simulink library "Lib_Piccolo"  (R2018b)
settings: Solver=VariableStepAuto  StartTime=0.0  StopTime=10.0  RelTol=1e-3
values from neighbouring files (symbols this model uses):
  AccelErrInt2Brakes = 0.15    [SimulationControlConfig16P.m]    (also in SimulationControlConfig16P_LEGACY.m; SimulationControlConfigTAILLESS.m = 0.2; SimulationControlConfigUTAIL.m = 0.2)
  AileronMax = 25    [SimulationControlConfig16P.m]    (also in SimulationControlConfig16P_LEGACY.m; SimulationControlConfigTAILLESS.m; SimulationControlConfigUTAIL.m)
  AileronPower = 0.00268    [SimulationControlConfig16P.m]    (also in SimulationControlConfig16P_LEGACY.m; SimulationControlConfigTAILLESS.m; SimulationControlConfigUTAIL.m)
  AileronSurfaceMax = 45    [SimulationControlConfig16P.m]    (also in SimulationControlConfig16P_LEGACY.m)
  AileronTrim = 0    [SimulationControlConfig16P.m]    (also in SimulationControlConfig16P_LEGACY.m; SimulationControlConfigTAILLESS.m; SimulationControlConfigUTAIL.m)
  Alt = 1000 + TerrainHeight    [SimulationStateConfig.m]
  AltCruise_m = testPlans(testIndx).terrainElevation * 0.3048 + 200    [SimulationControlConfig16P.m]    (also in SimulationControlConfigTAILLESS.m = 1083; SimulationControlConfigUTAIL.m = testPlans(testIndx).terrainElevation * 0.3048 + 152)
  AltitudeRate2PitchCmdIntegratorInit = 0.1    [SimulationControlPre.m]
  AltMax = 10000    [SimulationControlConfig16P.m]    (also in SimulationControlConfig16P_LEGACY.m; SimulationControlConfigTAILLESS.m; SimulationControlConfigUTAIL.m)
  AltMaxAccel = 1.25    [SimulationControlConfig16P.m]    (also in SimulationControlConfig16P_LEGACY.m = 0.9; SimulationControlConfigTAILLESS.m = 1.7; SimulationControlConfigUTAIL.m = 2)
  AltMin = 0    [SimulationControlConfig16P.m]    (also in SimulationControlConfig16P_LEGACY.m; SimulationControlConfigTAILLESS.m; SimulationControlConfigUTAIL.m)
  AltRateCmd2Pitch = 0.50    (= 0.5)    [SimulationControlConfig16P.m]    (also in SimulationControlConfig16P_LEGACY.m = 0.6; SimulationControlConfigTAILLESS.m = 0.2; SimulationControlConfigUTAIL.m = 0.3)
  AltRateError2Pitch = 0.40    (= 0.4)    [SimulationControlConfig16P.m]    (also in SimulationControlConfig16P_LEGACY.m; SimulationControlConfigTAILLESS.m = 0.55; SimulationControlConfigUTAIL.m = 0.55)
  AltRateErrorInt2Pitch = 0.50    (= 0.5)    [SimulationControlConfig16P.m]    (also in SimulationControlConfig16P_LEGACY.m = 0.45; SimulationControlConfigTAILLESS.m; SimulationControlConfigUTAIL.m = 0.75)
  AltRateLpfCutOff = 3    [SimulationControlConfig16P.m]    (also in SimulationControlConfig16P_LEGACY.m; SimulationControlConfigTAILLESS.m = 2; SimulationControlConfigUTAIL.m = 2)
  AutoNosegear2Rudder = 26    [SimulationControlConfig16P.m]    (also in SimulationControlConfig16P_LEGACY.m; SimulationControlConfigTAILLESS.m = 25.2; SimulationControlConfigUTAIL.m = 14)
  b = 5.54    [SimulationControlConfig16P.m]    (also in SimulationControlConfig16P_LEGACY.m; SimulationControlConfigTAILLESS.m = 2.37; SimulationControlConfigUTAIL.m = 2.37)
  Bank2AileronIntegratorInit = 0    [SimulationControlPre.m]
  BankMax_User = BankMax_User/180*pi    (= 0.523598775598)    [SimulationControlConfig16P.m]    (also in SimulationControlConfig16P_LEGACY.m; SimulationControlConfigTAILLESS.m = 0.610865238198; SimulationControlConfigUTAIL.m = 0.628318530718)
  baseLegFlaps = 20    [SimulationControlConfig16P.m]    (also in SimulationControlConfig16P_LEGACY.m = 0; SimulationControlConfigTAILLESS.m = 15; SimulationControlConfigUTAIL.m = 10)
  C = GeneticOpt.C    [SimulationCostFunction.m]
  c = Sw/b    (= 0.841696750903)    [SimulationControlConfig16P.m]    (also in SimulationControlConfig16P_LEGACY.m; SimulationControlConfigTAILLESS.m = 0.354008438819; SimulationControlConfigUTAIL.m = 0.354008438819)
  cell2WheelFactorMG = 5.98    [SimulationSensorConfig16P_LEGACY.m]
  cell2WheelFactorNG = 1    [SimulationSensorConfig16P_LEGACY.m]
  cellSatMaxMG = 15000    [SimulationSensorConfig16P.m]    (also in SimulationSensorConfig16P_LEGACY.m; SimulationSensorConfigTAILLESS7P.m; SimulationSensorConfigUTAIL7P.m)
  cellSatMaxNG = 1000    [SimulationSensorConfig16P.m]    (also in SimulationSensorConfig16P_LEGACY.m; SimulationSensorConfigTAILLESS7P.m; SimulationSensorConfigUTAIL7P.m)
  cellSatMinMG = -15000    [SimulationSensorConfig16P.m]    (also in SimulationSensorConfig16P_LEGACY.m; SimulationSensorConfigTAILLESS7P.m; SimulationSensorConfigUTAIL7P.m)
  cellSatMinNG = -1000    [SimulationSensorConfig16P.m]    (also in SimulationSensorConfig16P_LEGACY.m; SimulationSensorConfigTAILLESS7P.m; SimulationSensorConfigUTAIL7P.m)
  CL_Limit = CL_Max    (= 0.54)    [SimulationControlConfig16P.m]    (also in SimulationControlConfig16P_LEGACY.m; SimulationControlConfigTAILLESS.m; SimulationControlConfigUTAIL.m = 0.53)
  CL_Max = 0.54    [SimulationControlConfig16P.m]    (also in SimulationControlConfig16P_LEGACY.m; SimulationControlConfigTAILLESS.m; SimulationControlConfigUTAIL.m = 0.53)
  CL_Max_Nom = 0.465    [SimulationControlConfig16P.m]    (also in SimulationControlConfig16P_LEGACY.m; SimulationControlConfigTAILLESS.m = 0.39; SimulationControlConfigUTAIL.m)
  CL_Min = 0    [SimulationControlConfig16P.m]    (also in SimulationControlConfig16P_LEGACY.m; SimulationControlConfigTAILLESS.m; SimulationControlConfigUTAIL.m)
  ClimbMaxFraction = 0.35    [SimulationControlConfig16P.m]    (also in SimulationControlConfig16P_LEGACY.m = 0.24; SimulationControlConfigTAILLESS.m = 0.19; SimulationControlConfigUTAIL.m = 0.21)
  ClimboutMaxBank = 7.0    (= 7)    [SimulationControlConfig16P.m]    (also in SimulationControlConfig16P_LEGACY.m; SimulationControlConfigTAILLESS.m = 5; SimulationControlConfigUTAIL.m)
  ClimboutTimer = 7.0    (= 7)    [SimulationControlConfig16P.m]    (also in SimulationControlConfig16P_LEGACY.m; SimulationControlConfigTAILLESS.m; SimulationControlConfigUTAIL.m)
  dCl_per_dFlap = 0.005581818    [SimulationControlConfig16P.m]    (also in SimulationControlConfig16P_LEGACY.m = 0; SimulationControlConfigTAILLESS.m = 0; SimulationControlConfigUTAIL.m = 0)
  DecelerationCmd = 3.1    [SimulationControlConfig16P.m]    (also in SimulationControlConfig16P_LEGACY.m; SimulationControlConfigTAILLESS.m = 0.1; SimulationControlConfigUTAIL.m = 0.1)
  DeRotateLogicEndTimer = abs((NoseDownLimit_Deg-1)/DeRotateRamp_Dps)    [SimulationControlConfig16P.m]    (also in SimulationControlConfig16P_LEGACY.m; SimulationControlConfigTAILLESS.m; SimulationControlConfigUTAIL.m)
  DeRotateLogicHoldNoseUpTimer = 0.1    [SimulationControlConfig16P.m]    (also in SimulationControlConfig16P_LEGACY.m; SimulationControlConfigTAILLESS.m; SimulationControlConfigUTAIL.m)
  DeRotateLogicTimerTimeout = 2    [SimulationControlConfig16P.m]    (also in SimulationControlConfig16P_LEGACY.m; SimulationControlConfigTAILLESS.m; SimulationControlConfigUTAIL.m)
  DeRotateLowerCmdSaturation = 0    [SimulationControlConfig16P.m]    (also in SimulationControlConfig16P_LEGACY.m; SimulationControlConfigTAILLESS.m; SimulationControlConfigUTAIL.m)
  DeRotateRamp_Dps = 3    [SimulationControlConfig16P.m]    (also in SimulationControlConfig16P_LEGACY.m; SimulationControlConfigTAILLESS.m = 8; SimulationControlConfigUTAIL.m = 8)
  DeRotateUpperCmdSaturation = 7    [SimulationControlConfig16P.m]    (also in SimulationControlConfig16P_LEGACY.m; SimulationControlConfigTAILLESS.m; SimulationControlConfigUTAIL.m)
  DescentMaxFraction = 0.22    [SimulationControlConfig16P.m]    (also in SimulationControlConfig16P_LEGACY.m = 0.2; SimulationControlConfigTAILLESS.m = 0.17; SimulationControlConfigUTAIL.m = 0.17)
  DesktopSimTerrainOffset_m = 0.406    [SimulationAircraftConfig.m]
  downwindFlaps = 0    [SimulationControlConfig16P.m]    (also in SimulationControlConfig16P_LEGACY.m; SimulationControlConfigTAILLESS.m; SimulationControlConfigUTAIL.m)
  DP_init = 0.5*1.225*V_init^2    [SimulationControlConfig16P.m]    (also in SimulationControlConfig16P_LEGACY.m; SimulationControlConfigTAILLESS.m; SimulationControlConfigUTAIL.m)
  dscNoiseMG = 1    [SimulationSensorConfig16P_LEGACY.m]
  dscNoiseNG = 0.25    [SimulationSensorConfig16P_LEGACY.m]
  DSCnumBits = 24    [SimulationSensorConfig16P.m]    (also in SimulationSensorConfig16P_LEGACY.m; SimulationSensorConfigTAILLESS7P.m; SimulationSensorConfigUTAIL7P.m)
  DSCRangeMaxMG = 15000    [SimulationSensorConfig16P.m]    (also in SimulationSensorConfig16P_LEGACY.m; SimulationSensorConfigTAILLESS7P.m; SimulationSensorConfigUTAIL7P.m)
  DSCRangeMaxNG = 1000    [SimulationSensorConfig16P.m]    (also in SimulationSensorConfig16P_LEGACY.m; SimulationSensorConfigTAILLESS7P.m; SimulationSensorConfigUTAIL7P.m)
  DSCRangeMinMG = -15000    [SimulationSensorConfig16P.m]    (also in SimulationSensorConfig16P_LEGACY.m; SimulationSensorConfigTAILLESS7P.m; SimulationSensorConfigUTAIL7P.m)
  DSCRangeMinNG = -1000    [SimulationSensorConfig16P.m]    (also in SimulationSensorConfig16P_LEGACY.m; SimulationSensorConfigTAILLESS7P.m; SimulationSensorConfigUTAIL7P.m)
  dt = DLLSim.dt    [SimulationTimeStep.m]    (also in SimulationTrim.m = 0.02)
  EarlyTouchdownThreshold = 3.0    (= 3)    [SimulationControlConfig16P.m]    (also in SimulationControlConfig16P_LEGACY.m; SimulationControlConfigTAILLESS.m = 2.2; SimulationControlConfigUTAIL.m = 2.5)
  ElevatorDeflectionRate = 15    [SimulationControlConfig16P.m]    (also in SimulationControlConfig16P_LEGACY.m = 12; SimulationControlConfigTAILLESS.m = 10; SimulationControlConfigUTAIL.m = 12)
  ElevatorMax = 25    [SimulationControlConfig16P.m]    (also in SimulationControlConfig16P_LEGACY.m; SimulationControlConfigTAILLESS.m; SimulationControlConfigUTAIL.m)
  ElevatorPower = -0.002209    [SimulationControlConfig16P.m]    (also in SimulationControlConfig16P_LEGACY.m; SimulationControlConfigTAILLESS.m = -0.002956; SimulationControlConfigUTAIL.m = -0.00205983)
  ElevatorTrim = -3.5    [SimulationControlConfig16P.m]    (also in SimulationControlConfig16P_LEGACY.m; SimulationControlConfigTAILLESS.m = -6; SimulationControlConfigUTAIL.m = -8)
  elevonBias = 0    [SimulationControlConfig16P.m]    (also in SimulationControlConfig16P_LEGACY.m; SimulationControlConfigTAILLESS.m; SimulationControlConfigUTAIL.m)
  Enable_TAS_Protection = 0    [SimulationControlConfig16P.m]    (also in SimulationControlConfig16P_LEGACY.m; SimulationControlConfigTAILLESS.m; SimulationControlConfigUTAIL.m)
  EnableCrossTrackAbort = 1    [SimulationControlConfig16P.m]    (also in SimulationControlConfigTAILLESS.m; SimulationControlConfigUTAIL.m)
  EnergyBandwidth = 0.02    [SimulationControlConfig16P.m]    (also in SimulationControlConfig16P_LEGACY.m; SimulationControlConfigTAILLESS.m = 0.06; SimulationControlConfigUTAIL.m = 0.06)
  EngineLhFuelCut = 0    [SimulationAircraftConfig.m]
  EngineRhFuelCut = 0    [SimulationAircraftConfig.m]
  FastThrottleRate = 0.075    [SimulationControlConfig16P.m]    (also in SimulationControlConfig16P_LEGACY.m = 0.05; SimulationControlConfigTAILLESS.m = 0.1; SimulationControlConfigUTAIL.m = 0.1)
  FilterWarmUpTime = 2    [SimulationSensorConfig16P.m]    (also in SimulationSensorConfig16P_LEGACY.m; SimulationSensorConfigTAILLESS7P.m; SimulationSensorConfigUTAIL7P.m)
  finalApproachFlaps = 20    [SimulationControlConfig16P.m]    (also in SimulationControlConfig16P_LEGACY.m = 0; SimulationControlConfigTAILLESS.m = 22; SimulationControlConfigUTAIL.m = 10)
  FinalDescentSlope_Deg = testPlans(testIndx).descentSlope    [SimulationControlConfig16P.m]    (also in SimulationControlConfig16P_LEGACY.m; SimulationControlConfigTAILLESS.m; SimulationControlConfigUTAIL.m)
  flapMax = 0    [SimulationControlConfig16P.m]    (also in SimulationControlConfig16P_LEGACY.m; SimulationControlConfigTAILLESS.m; SimulationControlConfigUTAIL.m)
  flapRate = 7.5    [SimulationControlConfig16P.m]    (also in SimulationControlConfig16P_LEGACY.m; SimulationControlConfigTAILLESS.m = 6.6; SimulationControlConfigUTAIL.m)
  FlareHeight = 5    [SimulationControlConfig16P.m]    (also in SimulationControlConfig16P_LEGACY.m = 4.8; SimulationControlConfigTAILLESS.m = 2.5; SimulationControlConfigUTAIL.m = 2)
  FlareVerticalRate_mps = -0.4    [SimulationControlConfig16P.m]    (also in SimulationControlConfig16P_LEGACY.m = -0.5; SimulationControlConfigTAILLESS.m = -0.15; SimulationControlConfigUTAIL.m = -0.15)
  Fp_Aileron = 0.55*2*pi*RollRateLpfCutoff*dt    [SimulationControlConfig16P.m]    (also in SimulationControlConfig16P_LEGACY.m; SimulationControlConfigTAILLESS.m; SimulationControlConfigUTAIL.m)
  Fp_Alt = 0.55*AltBandwidth    (= 0.099)    [SimulationControlConfig16P.m]    (also in SimulationControlConfig16P_LEGACY.m; SimulationControlConfigTAILLESS.m = 0.587477826221; SimulationControlConfigUTAIL.m = 0.69115038379)
  Fp_AltRate = 0.55*2*pi*AltRateLpfCutOff*dt    [SimulationControlConfig16P.m]    (also in SimulationControlConfig16P_LEGACY.m; SimulationControlConfigTAILLESS.m; SimulationControlConfigUTAIL.m)
  Fp_Elevator = 0.55*2*pi*PitchRateLpfCutoff*dt    [SimulationControlConfig16P.m]    (also in SimulationControlConfig16P_LEGACY.m; SimulationControlConfigTAILLESS.m; SimulationControlConfigUTAIL.m)
  Fp_Energy = 0.55*2*pi*EnergyBandwidth    (= 0.069115038379)    [SimulationControlConfig16P.m]    (also in SimulationControlConfig16P_LEGACY.m; SimulationControlConfigTAILLESS.m = 0.207345115137; SimulationControlConfigUTAIL.m = 0.207345115137)
  Fp_Energy2 = 0.55*2*pi*EnergyBandwidth*dt    [SimulationControlConfig16P.m]    (also in SimulationControlConfig16P_LEGACY.m; SimulationControlConfigTAILLESS.m; SimulationControlConfigUTAIL.m)
  Fp_Pitch = 0.55*2*pi*PitchBandwidth    (= 2.76460153516)    [SimulationControlConfig16P.m]    (also in SimulationControlConfig16P_LEGACY.m = 3.11017672705; SimulationControlConfigTAILLESS.m = 3.80132711084; SimulationControlConfigUTAIL.m = 2.41902634326)
  Fp_Pitch_2 = 0.55*2*pi*PitchBandwidth*dt    [SimulationControlConfig16P.m]    (also in SimulationControlConfig16P_LEGACY.m; SimulationControlConfigTAILLESS.m; SimulationControlConfigUTAIL.m)
  Fp_Roll = RollBandwidth^2    (= 1)    [SimulationControlConfig16P.m]    (also in SimulationControlConfig16P_LEGACY.m = 1.44; SimulationControlConfigTAILLESS.m; SimulationControlConfigUTAIL.m)
  Fp_Rudder = 0.55*2*pi*YawRateLpfCutoff*dt    [SimulationControlConfig16P.m]    (also in SimulationControlConfig16P_LEGACY.m; SimulationControlConfigTAILLESS.m; SimulationControlConfigUTAIL.m)
  Fp_TAS = 0.55*2*pi*TASBandwidth    (= 0.103672557568)    [SimulationControlConfig16P.m]    (also in SimulationControlConfig16P_LEGACY.m; SimulationControlConfigTAILLESS.m = 0.172787595947; SimulationControlConfigUTAIL.m = 0.172787595947)
  Fp_TAS_Filter = 2*pi*TasLpfCutoff*dt    [SimulationControlConfig16P.m]    (also in SimulationControlConfig16P_LEGACY.m; SimulationControlConfigTAILLESS.m; SimulationControlConfigUTAIL.m)
  Fp_Turn = 0.55*2*pi*TurnErrLPFcutoff    (= 0.0345575191895)    [SimulationControlConfig16P.m]    (also in SimulationControlConfig16P_LEGACY.m; SimulationControlConfigTAILLESS.m = 0.172787595947; SimulationControlConfigUTAIL.m = 0.172787595947)
  Fp_TurnDerr = 0.55*2*pi*TurnDerivativeLPFcutoff    (= 0.0345575191895)    [SimulationControlConfig16P.m]    (also in SimulationControlConfig16P_LEGACY.m; SimulationControlConfigTAILLESS.m = 0.172787595947; SimulationControlConfigUTAIL.m = 0.172787595947)
  FTV = 3    [SimulationAircraftConfig.m]
  ftvStaticPositionError = 1/1.18    (= 0.847457627119)    [SimulationSensorConfig16P.m]    (also in SimulationSensorConfig16P_LEGACY.m; SimulationSensorConfigTAILLESS7P.m = 1; SimulationSensorConfigUTAIL7P.m = 1)
  g = 9.81    [SimulationStateConfig.m]
  GustSpd_Kts = testPlans(testIndx).gustSpd    [SimulationStateConfig.m]
  GustTriggerVal = testPlans(testIndx).gustTriggerVal    [SimulationStateConfig.m]
  HeadingErr2TurnRate = 0.5    [SimulationControlConfig16P.m]    (also in SimulationControlConfig16P_LEGACY.m; SimulationControlConfigTAILLESS.m; SimulationControlConfigUTAIL.m)
  HeadingErrDer2TurnRate = 0.3    [SimulationControlConfig16P.m]    (also in SimulationControlConfig16P_LEGACY.m; SimulationControlConfigTAILLESS.m; SimulationControlConfigUTAIL.m)
  IASbounce = IASstall*0.8    [SimulationControlPre.m]
  IAScruiseCMD = sqrt(2*m*9.81/(1.225*Sw*CL_cruise))    [SimulationControlConfig16P.m]    (also in SimulationControlConfig16P_LEGACY.m; SimulationControlConfigTAILLESS.m; SimulationControlConfigUTAIL.m)
  IASfinalCMD = 1.12 * IASmin    [SimulationControlConfig16P.m]    (also in SimulationControlConfig16P_LEGACY.m = 1.10 * IASmin; SimulationControlConfigTAILLESS.m = 1.10 * IASmin; SimulationControlConfigUTAIL.m = 1.15 * IASmin)
  IASflareCMD = IASstall    [SimulationControlConfig16P.m]    (also in SimulationControlConfig16P_LEGACY.m; SimulationControlConfigTAILLESS.m; SimulationControlConfigUTAIL.m)
  IASmax = 64    [SimulationControlConfig16P.m]    (also in SimulationControlConfig16P_LEGACY.m = 46; SimulationControlConfigTAILLESS.m = 38.58; SimulationControlConfigUTAIL.m = 35)
  IASmin = sqrt(2*m*9.81/(1.225*Sw*0.9*CL_Max_Nom))    [SimulationControlConfig16P.m]    (also in SimulationControlConfig16P_LEGACY.m; SimulationControlConfigTAILLESS.m; SimulationControlConfigUTAIL.m)
  IASshortCMD = IASstall    [SimulationControlConfig16P.m]    (also in SimulationControlConfig16P_LEGACY.m; SimulationControlConfigTAILLESS.m; SimulationControlConfigUTAIL.m)
  IASstall = sqrt(2*m*9.81/(1.225*Sw*CL_Max))    [SimulationControlConfig16P.m]    (also in SimulationControlConfig16P_LEGACY.m; SimulationControlConfigTAILLESS.m; SimulationControlConfigUTAIL.m)
  inFlight = 1    [SimulationControlConfig16P.m]    (also in SimulationControlConfigTAILLESS.m; SimulationControlConfigUTAIL.m)
  JetCatOffset = 5    [SimulationControlConfig16P.m]    (also in SimulationControlConfig16P_LEGACY.m)
  LaunchRollingElevator = -1.5    [SimulationControlConfig16P.m]    (also in SimulationControlConfig16P_LEGACY.m; SimulationControlConfigTAILLESS.m = 1; SimulationControlConfigUTAIL.m = 1)
  ldg_NosegearMax = 10    [SimulationControlConfig16P.m]    (also in SimulationControlConfig16P_LEGACY.m; SimulationControlConfigTAILLESS.m; SimulationControlConfigUTAIL.m)
  ldg_TrackVyErrInt2Nosegear = 0.1250    (= 0.125)    [SimulationControlConfig16P.m]    (also in SimulationControlConfig16P_LEGACY.m; SimulationControlConfigTAILLESS.m = 0.00714285714286; SimulationControlConfigUTAIL.m = 0.00714285714286)
  ldg_TrackVyErrPro2Nosegear = 0.35    [SimulationControlConfig16P.m]    (also in SimulationControlConfig16P_LEGACY.m; SimulationControlConfigTAILLESS.m = 0.0546666666667; SimulationControlConfigUTAIL.m = 0.0546666666667)
  ldg_TrackY2Vy = 0.07    [SimulationControlConfig16P.m]    (also in SimulationControlConfig16P_LEGACY.m; SimulationControlConfigTAILLESS.m = 0.17; SimulationControlConfigUTAIL.m = 0.17)
  ldg_Vy2NosegearScalingPower = 1.075    [SimulationControlConfig16P.m]    (also in SimulationControlConfig16P_LEGACY.m; SimulationControlConfigTAILLESS.m = 0.6; SimulationControlConfigUTAIL.m = 0.5)
  ldg_Y2VyScalingPower = 0.175    [SimulationControlConfig16P.m]    (also in SimulationControlConfig16P_LEGACY.m; SimulationControlConfigTAILLESS.m = 0; SimulationControlConfigUTAIL.m = 0)
  ldg_YawRate2Nosegear = 0.175    [SimulationControlConfig16P.m]    (also in SimulationControlConfig16P_LEGACY.m; SimulationControlConfigTAILLESS.m = 0.065; SimulationControlConfigUTAIL.m = 0.065)
  LiftSlope = 0.064285    [SimulationControlConfig16P.m]    (also in SimulationControlConfig16P_LEGACY.m; SimulationControlConfigTAILLESS.m = 0.058631; SimulationControlConfigUTAIL.m)
  LPFaileronInit = 0    [SimulationControlPre.m]
  LPFclestInit = 0    [SimulationControlPre.m]
  LPFenergyFFInit = 0    [SimulationControlPre.m]
  LPFtasInit = V_init + 2    [SimulationControlPre.m]
  LPFthrottleInit = ThrottleTrim    [SimulationControlPre.m]
  LPFturnErrInit = 0    [SimulationControlPre.m]
  ... (+115 more)
undefined symbols (not defined in the file or in its folder): abortFlag, alphaHPF, apmDelay, BRWNOUT, CRAWOR, CRAWUR, DiscIntNeverNeededParam, DLLSim, DLLSimStep, ECOMOR, ECOMUR, Fp_Tas, GustTrigger_HeightAgl_m, IPSTAT, LCINTEG, Ldg_Persist_Time, LOWER_FLAGS, MSG_ENABLE, NoiseStd, OLDVAL, OVERRIDE_ENABLE, OVERRIDE_VALUE, REBOOT, reversionEnable, revIASMax, revIASMin, revPitchMax, revPitchMin, revPitchRateMax, revRollMax, revRollRateMax, SAMPLE, SCALON, SensorModel, sigbuilder_block, Sim_Vx, Sim_Vy, Sim_Vz, Sim_Xpos, Sim_Ypos, Sim_Zpos, SYSOR, SYSUR, TARE, TEMPOR, TEMPUR, testIndx, testPlan, testPlans, Trim_piccoloInCmd, Trim_REFSI_FD_IN_nmodeCgShifterCmd_Ft, Trim_REFSI_FD_IN_nmodeFlapLhIBCmd_Deg, Trim_REFSI_FD_IN_nmodeFlapLhOBCmd_Deg, Trim_REFSI_FD_IN_nmodeFlapRhIBCmd_Deg, Trim_REFSI_FD_IN_nmodeFlapRhOBCmd_Deg, Trim_REFSI_FD_IN_nmodeSlatLhCmd_Deg, Trim_REFSI_FD_IN_nmodeSlatRhCmd_Deg, Trim_REFSI_FD_IN_nmodeSplrLhInbdCmd_Deg, Trim_REFSI_FD_IN_nmodeSplrLhOutbdCmd_Deg ... (+5)
libraries: simulink x866, aerolibconvert2 x60, $bdroot x52, aerolibatmos2 x5, dspswit3 x5, simulink_extras x4, dsparch4 x2, Lib_Piccolo_Alt x2, eeGeneralControl x1, dspindex x1
(part 8 of 44)

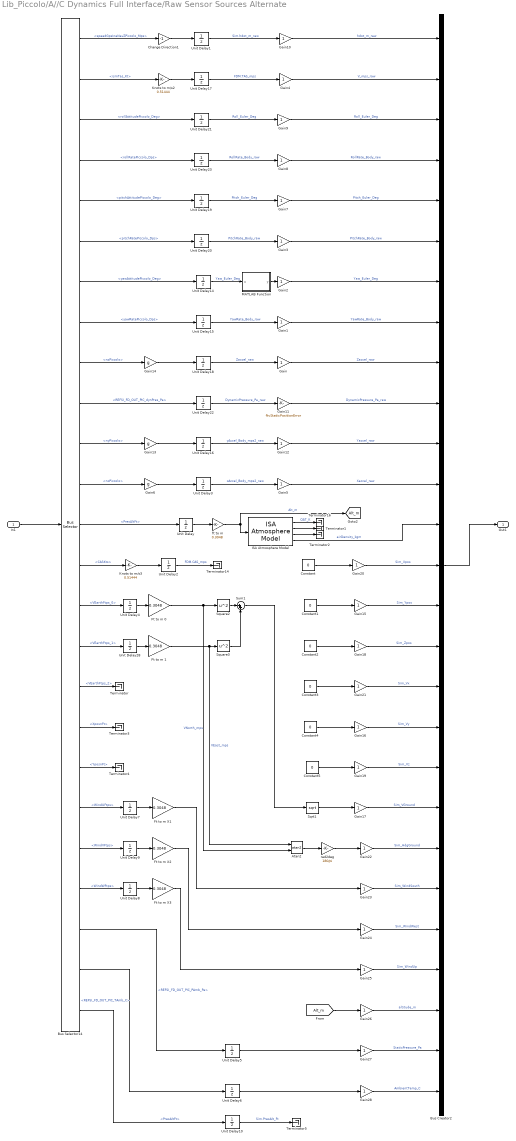
== system Lib_Piccolo/A//C Dynamics Full Interface/Raw Sensor Sources Alternate ==
  In1 : Inport
  Atan2 : Trigonometry  Operator=atan2
  Bus Creator2 : BusCreator  Inputs=27
  Bus Selector14 : BusSelector  OutputSignals=speedGpsIneNavZPiccolo_Mps,ismTas_Kt,rollAttitudePiccolo_Deg,rollRatePiccolo_Dps,pitchAttitudePiccolo_Deg,pitchRatePiccolo_Dps,yawAttitudePiccolo_Deg,yawRatePiccolo_Dps,nzPiccolo,REFSI_FD_OUT_PIC_dynPres_Pa,nyPiccolo,nxPiccolo,PresAltFt,CASKts,VEarthFtps_0,VEarthFtps_1,VEarthFtps_2,XposnFt,YposnFt,WindUFtps,WindVFtps,WindWFtps,REFSI_FD_OUT_PIC_PAmb_Pa,REFSI_FD_OUT_PIC_TAmb_C,PresAltFt
  Change Direction1 : Gain  Gain=-1
  Constant{,1..5} (6 alike) : Constant  Value=0
  Ft to m 0 : Gain  Gain=0.3048
  Ft to m 1 : Gain  Gain=0.3048
  Ft to m X1 : Gain  Gain=0.3048
  Ft to m X2 : Gain  Gain=0.3048
  Ft to m X3 : Gain  Gain=0.3048
  Gain{,1..5,7..10,12,15..28} (25 alike) : Gain
  Gain11 : Gain  Gain=ftvStaticPositionError
  Gain13 : Gain  Gain=g
  Gain14 : Gain  Gain=g
  Gain6 : Gain  Gain=g
  ISA Atmosphere Model : aerolibatmos2/ISA Atmosphere Model  custom=off  g=9.80665  gamma=1.4  R=287.0531  L=0.0065  h_trop=11000  h_strat=20000  rho0=1.225  P0=101325  T0=288.15  h0=0
      settings: SourceProductName=Aerospace Blockset
  Knots to m/s2 : Gain  Gain=0.51444
  Knots to m/s3 : Gain  Gain=0.51444
  MATLAB Function : MATLAB Function  TreatAsAtomicUnit=on
  Sqrt1 : Sqrt  OutputSignalType=real  SaturateOnIntegerOverflow=on
  Square2 : Math  Operator=square  OutputSignalType=real  SaturateOnIntegerOverflow=on
  Square3 : Math  Operator=square  OutputSignalType=real  SaturateOnIntegerOverflow=on
  Sum1 : Sum  Inputs=|++
  Terminator{,1..5,14,16} (8 alike) : Terminator
  Unit Delay : UnitDelay  InitialCondition=Alt  SampleTime=dt
  Unit Delay{1,3..4,7..9,15..16,20,23,28} (11 alike) : UnitDelay  SampleTime=-1
  Unit Delay10 : UnitDelay  InitialCondition=10  SampleTime=-1
  Unit Delay14 : UnitDelay  InitialCondition=SimObj.Output.PsiDeg  SampleTime=-1
  Unit Delay17 : UnitDelay  InitialCondition=V_init  SampleTime=-1
  Unit Delay18 : UnitDelay  InitialCondition=g  SampleTime=-1
  Unit Delay19 : UnitDelay  InitialCondition=SimObj.Output.ThetaDeg  SampleTime=-1
  Unit Delay2 : UnitDelay  InitialCondition=V_init  SampleTime=dt
  Unit Delay21 : UnitDelay  InitialCondition=SimObj.Output.PhiDeg  SampleTime=-1
  Unit Delay22 : UnitDelay  InitialCondition=DP_init  SampleTime=-1
  Unit Delay5 : UnitDelay  InitialCondition=90000  SampleTime=-1
  Unit Delay6 : UnitDelay  InitialCondition=10  SampleTime=-1
  ft to m : Gain  Gain=0.3048
  rad2deg : Gain  Gain=180/pi
  Out1 : Outport
  tag scope: Alt_m=global
  wires:
  Knots to m/s3/1 -> Unit Delay2/1
  Change Direction1/1 -> Unit Delay1/1
  Unit Delay23/1 -> Gain8/1  "RollRate_Body_raw"
  ISA Atmosphere Model/1 -> Terminator16/1  "OAT_K"
  Unit Delay22/1 -> Gain11/1  "DynamicPressure_Pa_raw"
  Unit Delay16/1 -> Gain12/1  "yAccel_Body_mps2_raw"
  Unit Delay17/1 -> Gain4/1  "FDM.TAS_mps"
  Unit Delay14/1 -> MATLAB Function/1(u)  "Yaw_Euler_Deg"
  ft to m/1 -> ISA Atmosphere Model/1, [Alt_m]  "Alt_m"
  Unit Delay2/1 -> Terminator14/1  "FDM.CAS_mps"
  Unit Delay18/1 -> Gain/1  "Zaccel_raw"
  Unit Delay20/1 -> Gain3/1  "PitchRate_Body_raw"
  Bus Selector14/13 -> Unit Delay/1  "<PresAltFt>"
  Unit Delay19/1 -> Gain7/1  "Pitch_Euler_Deg"
  Unit Delay15/1 -> Gain1/1  "YawRate_Body_raw"
  Unit Delay/1 -> ft to m/1
  Bus Selector14/14 -> Knots to m/s3/1  "<CASKts>"
  In1/1 -> Bus Selector14/1
  Gain4/1 -> Bus Creator2/2  "V_mps_raw"
  ISA Atmosphere Model/4 -> Bus Creator2/13  "airDensity_kgm"
  Knots to m/s2/1 -> Unit Delay17/1
  Unit Delay21/1 -> Gain9/1  "Roll_Euler_Deg"
  Bus Creator2/1 -> Out1/1
  ISA Atmosphere Model/2 -> Terminator1/1
  ISA Atmosphere Model/3 -> Terminator2/1
  Gain/1 -> Bus Creator2/9  "Zaccel_raw"
  Gain1/1 -> Bus Creator2/8  "YawRate_Body_raw"
  Gain2/1 -> Bus Creator2/7  "Yaw_Euler_Deg"
  Gain3/1 -> Bus Creator2/6  "PitchRate_Body_raw"
  Gain7/1 -> Bus Creator2/5  "Pitch_Euler_Deg"
  Gain8/1 -> Bus Creator2/4  "RollRate_Body_raw"
  Gain9/1 -> Bus Creator2/3  "Roll_Euler_Deg"
  Gain10/1 -> Bus Creator2/1  "hdot_m_raw"
  Gain11/1 -> Bus Creator2/10  "DynamicPressure_Pa_raw"
  Gain12/1 -> Bus Creator2/11  "Yaccel_raw"
  Bus Selector14/1 -> Change Direction1/1  "<speedGpsIneNavZPiccolo_Mps>"
  Bus Selector14/2 -> Knots to m/s2/1  "<ismTas_Kt>"
  Bus Selector14/3 -> Unit Delay21/1  "<rollAttitudePiccolo_Deg>"
  Bus Selector14/4 -> Unit Delay23/1  "<rollRatePiccolo_Dps>"
  Bus Selector14/5 -> Unit Delay19/1  "<pitchAttitudePiccolo_Deg>"
  Unit Delay1/1 -> Gain10/1  "Sim.hdot_m_raw"
  Bus Selector14/6 -> Unit Delay20/1  "<pitchRatePiccolo_Dps>"
  Bus Selector14/7 -> Unit Delay14/1  "<yawAttitudePiccolo_Deg>"
  Bus Selector14/8 -> Unit Delay15/1  "<yawRatePiccolo_Dps>"
  Bus Selector14/9 -> Gain14/1  "<nzPiccolo>"
  Bus Selector14/10 -> Unit Delay22/1  "<REFSI_FD_OUT_PIC_dynPres_Pa>"
  Bus Selector14/11 -> Gain13/1  "<nyPiccolo>"
  Bus Selector14/12 -> Gain6/1  "<nxPiccolo>"
  Unit Delay3/1 -> Gain5/1  "xAccel_Body_mps2_raw"
  Gain5/1 -> Bus Creator2/12  "Xaccel_raw"
  Gain6/1 -> Unit Delay3/1
  Gain13/1 -> Unit Delay16/1
  Gain14/1 -> Unit Delay18/1
  Bus Selector14/15 -> Unit Delay4/1  "<VEarthFtps_0>"
  Bus Selector14/16 -> Unit Delay28/1  "<VEarthFtps_1>"
  Unit Delay28/1 -> Ft to m 1/1
  Unit Delay4/1 -> Ft to m 0/1
  Bus Selector14/17 -> Terminator/1  "<VEarthFtps_2>"
  Gain15/1 -> Bus Creator2/15  "Sim_Ypos"
  Gain16/1 -> Bus Creator2/18  "Sim_Vy"
  Bus Selector14/18 -> Terminator3/1  "<XposnFt>"
  Sum1/1 -> Sqrt1/1
  Square2/1 -> Sum1/1
  Ft to m 0/1 -> Atan2/2, Square2/1  "VNorth_mps"
  Square3/1 -> Sum1/2
  Ft to m 1/1 -> Atan2/1, Square3/1  "VEast_mps"
  Gain17/1 -> Bus Creator2/20  "Sim_VGround"
  Gain18/1 -> Bus Creator2/16  "Sim_Zpos"
  Gain19/1 -> Bus Creator2/19  "Sim_Vz"
  Gain20/1 -> Bus Creator2/14  "Sim_Xpos"
  Gain21/1 -> Bus Creator2/17  "Sim_Vx"
  Gain22/1 -> Bus Creator2/21  "Sim_HdgGround"
  Gain23/1 -> Bus Creator2/22  "Sim_WindSouth"
  Gain24/1 -> Bus Creator2/23  "Sim_WindWest"
  Constant/1 -> Gain20/1
  Constant1/1 -> Gain15/1
  Constant2/1 -> Gain18/1
  Constant3/1 -> Gain21/1
  Constant4/1 -> Gain16/1
  Constant5/1 -> Gain19/1
  Sqrt1/1 -> Gain17/1
  Ft to m X1/1 -> Gain23/1
  Ft to m X2/1 -> Gain24/1
  Ft to m X3/1 -> Gain25/1
  Gain25/1 -> Bus Creator2/24  "Sim_WindUp"
  Bus Selector14/20 -> Unit Delay7/1  "<WindUFtps>"
  Bus Selector14/21 -> Unit Delay9/1  "<WindVFtps>"
  Bus Selector14/22 -> Unit Delay8/1  "<WindWFtps>"
  Unit Delay7/1 -> Ft to m X1/1
  Unit Delay9/1 -> Ft to m X2/1
  Unit Delay8/1 -> Ft to m X3/1
  Atan2/1 -> rad2deg/1
  rad2deg/1 -> Gain22/1
  Bus Selector14/19 -> Terminator4/1  "<YposnFt>"
  Gain26/1 -> Bus Creator2/25  "altitude_m"
  [Alt_m] -> Gain26/1
  MATLAB Function/1(y) -> Gain2/1
  Bus Selector14/23 -> Unit Delay5/1  "<REFSI_FD_OUT_PIC_PAmb_Pa>"
  Unit Delay5/1 -> Gain27/1
  Gain27/1 -> Bus Creator2/26  "StaticPressure_Pa"
  Unit Delay6/1 -> Gain28/1
  Bus Selector14/24 -> Unit Delay6/1  "<REFSI_FD_OUT_PIC_TAmb_C>"
  Gain28/1 -> Bus Creator2/27  "AmbientTemp_C"
  Bus Selector14/25 -> Unit Delay10/1  "<PresAltFt>"
  Unit Delay10/1 -> Terminator5/1  "Sim.PresAlt_Ft"

== system Lib_Piccolo/A//C Dynamics Full Interface/Raw Sensor Sources Jack ==
  In1 : Inport
  Bus Creator2 : BusCreator  Inputs=12
  Bus Selector14 : BusSelector  OutputSignals=VEarthFtps_2,TASKts,PhiDeg,PDps,ThetaDeg,QDps,PsiDeg,RDps,NzG,REFSI_FD_OUT_PIC_dynPres_Pa,NyG,AlphaDeg,NxG,GrndContactNG,GrndContactLMG,GrndContactRMG,PresAltFt,CASKts
  Change Direction1 : Gain  Gain=-1
  Ft to m1 : Gain  Gain=0.3048
  Gain4 : Gain
  Gain5 : Gain  Gain=g
  Gain6 : Gain  Gain=g
  ISA Atmosphere Model : aerolibatmos2/ISA Atmosphere Model  custom=off  g=9.80665  gamma=1.4  R=287.0531  L=0.0065  h_trop=11000  h_strat=20000  rho0=1.225  P0=101325  T0=288.15  h0=0
      settings: SourceProductName=Aerospace Blockset
  Knots to m/s2 : Gain  Gain=0.51444
  Knots to m/s3 : Gain  Gain=0.51444
  Scope4 : Scope  NumInputPorts=2
  Terminator{,1..5,14,16} (8 alike) : Terminator
  Unit Delay : UnitDelay  InitialCondition=Alt  SampleTime=dt
  Unit Delay14 : UnitDelay  InitialCondition=SimObj.Output.PsiDeg  SampleTime=-1
  Unit Delay{15..16,20,23} (4 alike) : UnitDelay  SampleTime=-1
  Unit Delay17 : UnitDelay  InitialCondition=V_init  SampleTime=-1
  Unit Delay18 : UnitDelay  InitialCondition=1  SampleTime=-1
  Unit Delay19 : UnitDelay  InitialCondition=SimObj.Output.ThetaDeg  SampleTime=-1
  Unit Delay2 : UnitDelay  InitialCondition=V_init  SampleTime=dt
  Unit Delay21 : UnitDelay  InitialCondition=SimObj.Output.PhiDeg  SampleTime=-1
  Unit Delay22 : UnitDelay  InitialCondition=DP_init  SampleTime=-1
  ft to m : Gain  Gain=0.3048
  Out1 : Outport
  wires:
  Knots to m/s3/1 -> Unit Delay2/1
  Ft to m1/1 -> Bus Creator2/1  "hdot_m_raw"
  Unit Delay23/1 -> Bus Creator2/4  "RollRate_Body_raw"
  ISA Atmosphere Model/1 -> Terminator16/1  "OAT_K"
  Unit Delay22/1 -> Bus Creator2/10  "DynamicPressure_Pa_raw"
  Unit Delay16/1 -> Gain5/1  "yAccel_Body_mps2_raw"
  Bus Selector14/6 -> Unit Delay20/1  "<QDps>"
  Bus Selector14/7 -> Unit Delay14/1  "<PsiDeg>"
  Unit Delay17/1 -> Gain4/1  "Sim.TAS"
  Bus Selector14/4 -> Unit Delay23/1  "<PDps>"
  Bus Selector14/9 -> Unit Delay18/1  "<NzG>"
  Bus Selector14/1 -> Change Direction1/1  "<VEarthFtps_2>"
  Unit Delay14/1 -> Bus Creator2/7  "Yaw_Euler_Deg"
  ft to m/1 -> ISA Atmosphere Model/1  "Alt_m"
  Unit Delay2/1 -> Terminator14/1  "CAS_mps"
  Change Direction1/1 -> Ft to m1/1
  Unit Delay18/1 -> Gain6/1  "NzG_raw (g)"
  Unit Delay20/1 -> Bus Creator2/6  "PitchRate_Body_raw"
  Bus Selector14/8 -> Unit Delay15/1  "<RDps>"
  Bus Selector14/17 -> Unit Delay/1  "<PresAltFt>"
  Unit Delay19/1 -> Bus Creator2/5  "Pitch_Euler_Deg"
  Unit Delay15/1 -> Bus Creator2/8  "YawRate_Body_raw"
  Bus Selector14/12 -> Scope4/1  "<AlphaDeg>"
  Unit Delay/1 -> ft to m/1
  Bus Selector14/2 -> Knots to m/s2/1  "<TASKts>"
  Gain6/1 -> Bus Creator2/9  "Zaccel_raw"
  Bus Selector14/18 -> Knots to m/s3/1  "<CASKts>"
  In1/1 -> Bus Selector14/1
  Bus Selector14/13 -> Terminator/1  "<NxG>"
  Bus Selector14/11 -> Unit Delay16/1  "<NyG>"
  [AoA] -> Scope4/2
  Bus Selector14/10 -> Unit Delay22/1  "<REFSI_FD_OUT_PIC_dynPres_Pa>"
  Gain5/1 -> Bus Creator2/11  "Yaccel_raw"
  Gain4/1 -> Bus Creator2/2  "V_mps_raw"
  ISA Atmosphere Model/4 -> Bus Creator2/12  "airDensity_kgm"
  Knots to m/s2/1 -> Unit Delay17/1
  Unit Delay21/1 -> Bus Creator2/3  "Roll_Euler_Deg"
  Bus Selector14/5 -> Unit Delay19/1  "<ThetaDeg>"
  Bus Selector14/3 -> Unit Delay21/1  "<PhiDeg>"
  Bus Creator2/1 -> Out1/1
  ISA Atmosphere Model/2 -> Terminator1/1
  ISA Atmosphere Model/3 -> Terminator2/1
  Bus Selector14/16 -> Terminator5/1  "<GrndContactRMG>"
  Bus Selector14/15 -> Terminator4/1  "<GrndContactLMG>"
  Bus Selector14/14 -> Terminator3/1  "<GrndContactNG>"

== system Lib_Piccolo/A//C Dynamics Full Interface/SIM Exit Conditions ==
  In1 : Inport
  AND : Logic  IconShape=distinctive  AllPortsSameDT=off  OutDataTypeStr=boolean
  Bus Selector14 : BusSelector  OutputSignals=GrndContactNG,GrndContactLMG,GrndContactRMG,VEarthFtps_0,VEarthFtps_1
  Clock : Clock
  Compare To Constant : simulink/Logic and Bit Operations/Compare To Constant  relop=<=  const=0.01  OutDataTypeStr=boolean
  Compare To Constant1 : simulink/Logic and Bit Operations/Compare To Constant  relop=>  const=15  OutDataTypeStr=boolean
  Ft to m 0 : Gain  Gain=0.3048
  Ft to m 1 : Gain  Gain=0.3048
  Manual Switch : ManualSwitch
  OR3 : Logic  Operator=OR  IconShape=distinctive  AllPortsSameDT=off  OutDataTypeStr=boolean
  OR4 : Logic  Operator=OR  IconShape=distinctive  AllPortsSameDT=off  OutDataTypeStr=boolean
  Sqrt1 : Sqrt  OutputSignalType=real  SaturateOnIntegerOverflow=on
  Square2 : Math  Operator=square  OutputSignalType=real  SaturateOnIntegerOverflow=on
  Square3 : Math  Operator=square  OutputSignalType=real  SaturateOnIntegerOverflow=on
  Stop Simulation : Stop  Commented=on
  Stop Simulation1 : Stop
  Sum1 : Sum  Inputs=|++
  Timer : Subsystem  mask{period=10}
      mask prompts: period "Period [s]"
  wires:
  Timer/1(Expired) -> Manual Switch/1
  OR3/1 -> OR4/1
  Bus Selector14/3 -> OR4/2  "<GrndContactRMG>"
  OR4/1 -> Timer/1(Enable/!Rst), Manual Switch/2
  Bus Selector14/2 -> OR3/2  "<GrndContactLMG>"
  In1/1 -> Bus Selector14/1
  Bus Selector14/1 -> OR3/1  "<GrndContactNG>"
  Manual Switch/1 -> Stop Simulation/1
  AND/1 -> Stop Simulation1/1
  Compare To Constant/1 -> AND/1
  Compare To Constant1/1 -> AND/2
  Sqrt1/1 -> Compare To Constant/1  "Sim_VGround"
  Clock/1 -> Compare To Constant1/1
  Ft to m 0/1 -> Square2/1  "VNorth_mps"
  Ft to m 1/1 -> Square3/1  "VEast_mps"
  Square3/1 -> Sum1/2
  Square2/1 -> Sum1/1
  Sum1/1 -> Sqrt1/1
  Bus Selector14/5 -> Ft to m 1/1  "<VEarthFtps_1>"
  Bus Selector14/4 -> Ft to m 0/1  "<VEarthFtps_0>"

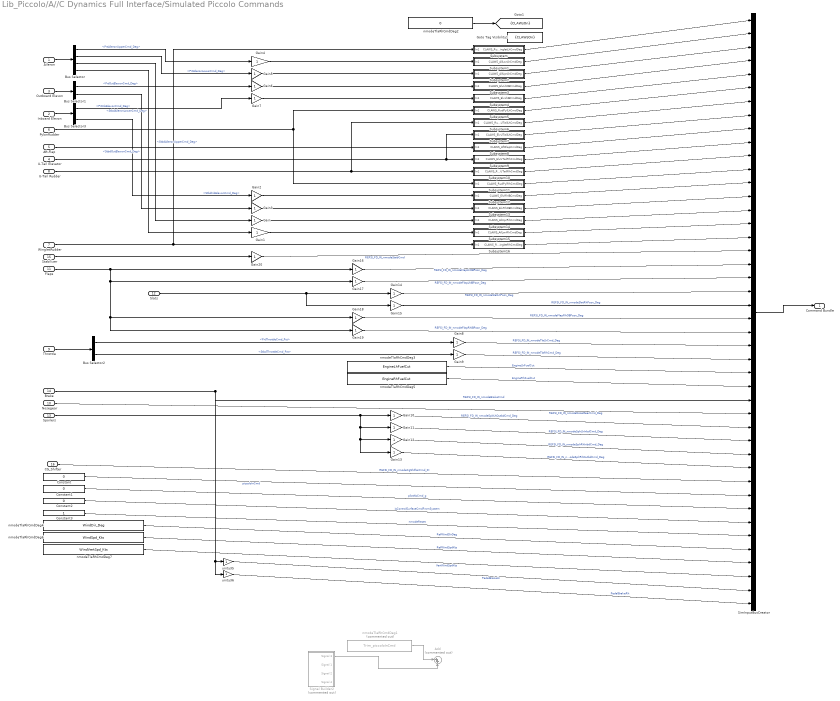
== system Lib_Piccolo/A//C Dynamics Full Interface/Simulated Piccolo Commands ==
  Aileron : Inport
  Inboard Elevon : Inport  Port=2
  Outboard Elevon : Inport  Port=3
  U-Tail Elevator : Inport  Port=4
  Aft-Flap : Inport  Port=5
  "PylonRudder " : Inport  Port=6
  "WingletRudder " : Inport  Port=7
  U-Tail Rudder : Inport  Port=8
  "Throttle " : Inport  Port=9
  Nosegear : Inport  Port=10
  Flaps : Inport  Port=11
  Slats : Inport  Port=12
  Spoilers : Inport  Port=13
  Brake : Inport  Port=14
  Stabilizer : Inport  Port=15
  CG_Shifter : Inport  Port=16
  Add : Sum  Commented=on  Inputs=|++
  Bus Selector : BusSelector  OutputSignals=PrtAileronUpperCmd_Deg,PrtAileronLowerCmd_Deg,StbdAileronUpperCmd_Deg,StbdAileronLowerCmd_Deg
  Bus Selector1 : BusSelector  OutputSignals=PrtOutElevonCmd_Deg,StbdOutElevonCmd_Deg
  Bus Selector2 : BusSelector  OutputSignals=PrtThrottleCmd_Pct,StbdThrottleCmd_Pct
  Bus Selector3 : BusSelector  OutputSignals=PrtInbElevonCmd_Deg,StbdInbElevonCmd_Deg
  Constant : Constant  Value=0
  Constant1 : Constant  Value=0
  Constant2 : Constant  Value=0
  Constant3 : Constant
  Gain{,1..20} (21 alike) : Gain
  Goto Tag Visibility1 : GotoTagVisibility  GotoTag=CLAWsOn
  Signal Builder2 : Subsystem  Tag=STV Subsys  Commented=on  LoadFcn=sigbuilder_block('load');  StartFcn=sigbuilder_block('start');  StopFcn=sigbuilder_block('stop');  ClipboardFcn=sigbuilder_block('clipboard');  mask(Sigbuilder block){tuvar=[0:10]}
      mask help: Simulink:masks:SigbuilderBlock_MD
      mask init:
      | if ~strcmp(get_param(bdroot(gcbh),'SimulationStatus'),'stopped') tuvar = sigbuilder_block('maskInit'); end
      settings: CopyFcn=sigbuilder_block('copy');  DeleteFcn=sigbuilder_block('delete');  ModelCloseFcn=sigbuilder_block('modelClose');  PreSaveFcn=sigbuilder_block('preSave');  PauseFcn=sigbuilder_block('pause');  ContinueFcn=sigbuilder_block('continue');  NameChangeFcn=sigbuilder_block('namechange');  OpenFcn=sigbuilder_block('open',[421.8 380.4 544.2 313.2 ]);  CloseFcn=sigbuilder_block('close');
      mask Display: plot(0, 0, 100, 100,[2, 2, 32, 32, 2], [68, 8, 8, 68, 68],[32, 2], [38, 38], [32, 19, 2],[53, 60, 44], [32, 17, 17, 2],[16, 16, 31, 31]);txt = getActiveGroup(gcbh);text(2, 100, txt,'verticalAlignment', 'top');
  SimInputBusCreator : BusCreator  Inputs=44
  Subsystem : Subsystem
  Subsystem1 : Subsystem
  Subsystem10 : Subsystem
  Subsystem11 : Subsystem
  Subsystem12 : Subsystem
  Subsystem13 : Subsystem
  Subsystem14 : Subsystem
  Subsystem15 : Subsystem
  Subsystem16 : Subsystem
  Subsystem2 : Subsystem
  Subsystem3 : Subsystem
  Subsystem4 : Subsystem
  Subsystem5 : Subsystem
  Subsystem6 : Subsystem
  Subsystem7 : Subsystem
  Subsystem8 : Subsystem
  Subsystem9 : Subsystem
  nmodeTlaRhCmdDeg1 : Constant  Commented=on  Value=Trim_piccoloInCmd
  nmodeTlaRhCmdDeg2 : Constant  Value=0
  nmodeTlaRhCmdDeg3 : Constant  Value=EngineLhFuelCut
  nmodeTlaRhCmdDeg4 : Constant  Value=WindDir_Deg
  nmodeTlaRhCmdDeg5 : Constant  Value=EngineRhFuelCut
  nmodeTlaRhCmdDeg6 : Constant  Value=WindSpd_Kts
  nmodeTlaRhCmdDeg7 : Constant  Value=WindVertSpd_Kts
  unity35 : Gain
  unity36 : Gain
  Command Bundle : Outport
  tag scope: CLAWsOn=scoped
  wires:
  nmodeTlaRhCmdDeg7/1 -> SimInputBusCreator/42  "VertWindSpdKts"
  Gain20/1 -> SimInputBusCreator/18  "REFSI_FD_IN_nmodeStabCmd"
  Subsystem4/1(CLAWS_ElvLhIBCmdDeg) -> SimInputBusCreator/5
  Subsystem/1(CLAWS_RudWingletLhCmdDeg) -> SimInputBusCreator/1
  nmodeTlaRhCmdDeg3/1 -> SimInputBusCreator/27  "EngineLhFuelCut"
  Subsystem2/1(CLAWS_AilUprLhCmdDeg) -> SimInputBusCreator/3
  Gain15/1 -> SimInputBusCreator/22  "REFSI_FD_IN_nmodeSlatRhPosn_Deg"
  Gain14/1 -> SimInputBusCreator/21  "REFSI_FD_IN_nmodeSlatLhPosn_Deg"
  Subsystem10/1(CLAWS_RudUTailRhCmdDeg) -> SimInputBusCreator/11
  Subsystem14/1(CLAWS_AilUprRhCmdDeg) -> SimInputBusCreator/15
  Subsystem6/1(CLAWS_RudUTailLhCmdDeg) -> SimInputBusCreator/7
  Subsystem5/1(CLAWS_RudPylLhCmdDeg) -> SimInputBusCreator/6
  Subsystem8/1(CLAWS_AftFlapCmdDeg) -> SimInputBusCreator/9
  Nosegear/1 -> SimInputBusCreator/30  "REFSI_FD_IN_nmodeNoseGearCmd_Deg"
  Subsystem12/1(CLAWS_ElvRhIBCmdDeg) -> SimInputBusCreator/13
  Subsystem16/1(CLAWS_RudWingletRhCmdDeg) -> SimInputBusCreator/17
  Gain10/1 -> SimInputBusCreator/31  "REFSI_FD_IN_nmodeSplrLhOutbdCmd_Deg"
  nmodeTlaRhCmdDeg2/1 -> [CLAWsOn]
  Subsystem13/1(CLAWS_ElvRhOBCmdDeg) -> SimInputBusCreator/14
  Aft-Flap/1 -> Subsystem8/1(In1)
  Signal Builder2/1(Signal 3) -> Add/2
  nmodeTlaRhCmdDeg1/1 -> Add/1
  Subsystem11/1(CLAWS_RudPylRhCmdDeg) -> SimInputBusCreator/12
  "PylonRudder "/1 -> Subsystem11/1(In1), Subsystem5/1(In1)
  Gain18/1 -> SimInputBusCreator/23  "REFSI_FD_IN_nmodeFlapRhOBPosn_Deg"
  Subsystem9/1(CLAWS_ElvUTailRhCmdDeg) -> SimInputBusCreator/10
  Gain13/1 -> SimInputBusCreator/34  "REFSI_FD_IN_nmodeSplrRhOutbdCmd_Deg"
  nmodeTlaRhCmdDeg5/1 -> SimInputBusCreator/28  "EngineRhFuelCut"
  Gain17/1 -> SimInputBusCreator/20  "REFSI_FD_IN_nmodeFlapLhIBPosn_Deg"
  U-Tail Rudder/1 -> Subsystem10/1(In1), Subsystem6/1(In1)
  Gain19/1 -> SimInputBusCreator/24  "REFSI_FD_IN_nmodeFlapRhIBPosn_Deg"
  Gain16/1 -> SimInputBusCreator/19  "REFSI_FD_IN_nmodeFlapLhOBPosn_Deg"
  Subsystem1/1(CLAWS_AilLwrLhCmdDeg) -> SimInputBusCreator/2
  "WingletRudder "/1 -> Subsystem/1(In1), Subsystem16/1(In1)
  Subsystem3/1(CLAWS_ElvLhOBCmdDeg) -> SimInputBusCreator/4
  Subsystem7/1(CLAWS_ElvUTailLhCmdDeg) -> SimInputBusCreator/8
  Gain12/1 -> SimInputBusCreator/33  "REFSI_FD_IN_nmodeSplrRhInbdCmd_Deg"
  Subsystem15/1(CLAWS_AilLwrRhCmdDeg) -> SimInputBusCreator/16
  CG_Shifter/1 -> SimInputBusCreator/35  "REFSI_FD_IN_nmodeCgShifterCmd_Ft"
  Gain11/1 -> SimInputBusCreator/32  "REFSI_FD_IN_nmodeSplrLhInbdCmd_Deg"
  Brake/1 -> unity36/1, unity35/1, SimInputBusCreator/29  "REFSI_FD_IN_nmodeBrakeCmd"
  U-Tail Elevator/1 -> Subsystem9/1(In1), Subsystem7/1(In1)
  SimInputBusCreator/1 -> Command Bundle/1
  Gain/1 -> Subsystem14/1(In1)
  Gain1/1 -> Subsystem15/1(In1)
  Gain2/1 -> Subsystem12/1(In1)
  Gain3/1 -> Subsystem13/1(In1)
  Gain4/1 -> Subsystem1/1(In1)
  Gain5/1 -> Subsystem2/1(In1)
  Gain6/1 -> Subsystem3/1(In1)
  Gain7/1 -> Subsystem4/1(In1)
  Constant1/1 -> SimInputBusCreator/37  "pilotNzCmd_g"
  Constant/1 -> SimInputBusCreator/36  "piccoloInCmd"
  Constant2/1 -> SimInputBusCreator/38  "isControlSurfaceCmdFromSystem"
  Constant3/1 -> SimInputBusCreator/39  "nmodeReset"
  nmodeTlaRhCmdDeg4/1 -> SimInputBusCreator/40  "RefWindDirDeg"
  nmodeTlaRhCmdDeg6/1 -> SimInputBusCreator/41  "RefWindSpdKts"
  unity36/1 -> SimInputBusCreator/44  "PedalBrakeRh"
  unity35/1 -> SimInputBusCreator/43  "PedalBrakeLh"
  Gain8/1 -> SimInputBusCreator/25  "REFSI_FD_IN_nmodeTlaLhCmd_Deg"
  Gain9/1 -> SimInputBusCreator/26  "REFSI_FD_IN_nmodeTlaRhCmd_Deg"
  Aileron/1 -> Bus Selector/1
  Bus Selector/1 -> Gain4/1  "<PrtAileronUpperCmd_Deg>"
  Bus Selector/2 -> Gain5/1  "<PrtAileronLowerCmd_Deg>"
  Bus Selector/3 -> Gain/1  "<StbdAileronUpperCmd_Deg>"
  Bus Selector/4 -> Gain1/1  "<StbdAileronLowerCmd_Deg>"
  Outboard Elevon/1 -> Bus Selector1/1
  Bus Selector1/1 -> Gain6/1  "<PrtOutElevonCmd_Deg>"
  Bus Selector1/2 -> Gain3/1  "<StbdOutElevonCmd_Deg>"
  "Throttle "/1 -> Bus Selector2/1
  Bus Selector2/1 -> Gain8/1  "<PrtThrottleCmd_Pct>"
  Bus Selector2/2 -> Gain9/1  "<StbdThrottleCmd_Pct>"
  Inboard Elevon/1 -> Bus Selector3/1
  Bus Selector3/1 -> Gain7/1  "<PrtInbElevonCmd_Deg>"
  Bus Selector3/2 -> Gain2/1  "<StbdInbElevonCmd_Deg>"
  Spoilers/1 -> Gain13/1, Gain12/1, Gain11/1, Gain10/1
  Slats/1 -> Gain15/1, Gain14/1
  Flaps/1 -> Gain19/1, Gain18/1, Gain17/1, Gain16/1
  Stabilizer/1 -> Gain20/1

== system Lib_Piccolo/APM State Limits/Latch ==
  D : Inport
  Enable/!Rst : Inport  Port=2
  AND : Logic  IconShape=distinctive  AllPortsSameDT=off  OutDataTypeStr=boolean
  Constant : Constant
  OR : Logic  Operator=OR  IconShape=distinctive  AllPortsSameDT=off  OutDataTypeStr=boolean
  Switch : Switch  Criteria=u2 > Threshold  Threshold=0.5
  Unit Delay : UnitDelay  SampleTime=-1
  Q_Latched : Outport
  wires:
  Unit Delay/1 -> OR/2
  Switch/1 -> Q_Latched/1, Unit Delay/1
  D/1 -> Switch/3, OR/1
  OR/1 -> AND/1
  AND/1 -> Switch/2
  Enable/!Rst/1 -> AND/2
  Constant/1 -> Switch/1

== system Lib_Piccolo/Airspeed Complementary Filter/HPF Acceleration ==
  note: "Approximated" HPF, x - LPF(x) = HPF(x)
  note: "True" IIR HPF (not used, but for reference)
  note: Implements the High Pass Difference Equation:
      |
      | $y[n] = \frac {1+\alpha}2 \cdot (x[n] -x[n-1]) + \alpha \cdot y[n-1]$
  Input : Inport
  Gain : Gain  Commented=on  Gain=(1+alphaHPF)/2
  Gain1 : Gain  Commented=on  Gain=alphaHPF
  LFP Nx : Subsystem
  Sum : Sum  Inputs=+-|
  Sum2 : Sum  Commented=on  Inputs=++|
  Sum3 : Sum  Commented=on  Inputs=|+-
  Terminator : Terminator  Commented=on
  Unit Delay1 : UnitDelay  Commented=on  SampleTime=-1
  Unit Delay2 : UnitDelay  Commented=on  SampleTime=-1
  Output : Outport
  wires:
  Input/1 -> LFP Nx/1(Input), Sum/1, Sum3/1, Unit Delay1/1  "x_n"
  Gain1/1 -> Sum2/1
  Gain/1 -> Sum2/2
  Unit Delay1/1 -> Sum3/2  "x_n-1"
  Sum2/1 -> Terminator/1, Unit Delay2/1  "y_n"
  Sum3/1 -> Gain/1
  Unit Delay2/1 -> Gain1/1  "y_n-1"
  LFP Nx/1(Output) -> Sum/2
  Sum/1 -> Output/1

== system Lib_Piccolo/Airspeed Complementary Filter/LPF TAS ==
  Input : Inport
  Reset : Inport  Port=2
  Add1 : Sum  Inputs=++|
  Compare To Constant2 : simulink/Logic and Bit Operations/Compare To Constant  relop=>  const=0  OutDataTypeStr=uint8
  Constant11 : Constant  Value=TasLpfCutoff
  Switch1 : Switch  Criteria=u2 > Threshold
  Unit Delay1 : UnitDelay  InitialCondition=LPFtasInit  SampleTime=-1
  a1 : Gain  Gain=1-Fp_TAS_Filter
  b0 : Gain  Gain=Fp_TAS_Filter
  Output : Outport
  wires:
  Constant11/1 -> Compare To Constant2/1
  Compare To Constant2/1 -> Switch1/2
  Switch1/1 -> Output/1
  Input/1 -> b0/1, Switch1/3
  Add1/1 -> Switch1/1, Unit Delay1/1
  a1/1 -> Add1/1
  b0/1 -> Add1/2
  Unit Delay1/1 -> a1/1

== system Lib_Piccolo/Airspeed Reference Model/Airspeed Control Only Used In Airspeed Mode ==
  "Vcmd " : Inport
  Feedback Bus : Inport  Port=2
  Bus Selector : BusSelector  OutputSignals=V_mps
  Gain : Gain  Gain=Fp_TAS
  "Saturation " : Saturate  UpperLimit=TASRateMax  LowerLimit=-TASRateMax
  Sum : Sum  Inputs=|+-
  Sum1 : Sum  Inputs=|++
  "VdotCmd " : Constant  Value=0
  VdotCmd : Outport
  tag scope: TASErr=global
  wires:
  "Vcmd "/1 -> Sum/1
  Sum/1 -> [TASErr], Gain/1
  Gain/1 -> Sum1/1
  "VdotCmd "/1 -> Sum1/2
  Sum1/1 -> "Saturation "/1
  "Saturation "/1 -> VdotCmd/1  "Sim.TASRateCmd (airspeed)"
  Feedback Bus/1 -> Bus Selector/1
  Bus Selector/1 -> Sum/2  "<V_mps>"

== system Lib_Piccolo/Airspeed Reference Model/TAS Rate to Altitude Rate Command ==
  VdotCmd : Inport
  Feedback Bus : Inport  Port=2
  Vcmd : Inport  Port=3
  Bus Selector : BusSelector  OutputSignals=Vdot_mps2,V_mps,apMode
  Compare To Constant : simulink/Logic and Bit Operations/Compare To Constant  relop=<=  const=3  OutDataTypeStr=boolean
  NOT : Logic  Operator=NOT  IconShape=distinctive  AllPortsSameDT=off  OutDataTypeStr=boolean
  NOT1 : Logic  Operator=NOT  IconShape=distinctive  AllPortsSameDT=off  OutDataTypeStr=boolean
  OR : Logic  Operator=OR  Inputs=3  IconShape=distinctive  AllPortsSameDT=off  OutDataTypeStr=boolean
  PID Controller : simulink/Continuous/PID Controller  Controller=PID  Form=Parallel  TimeDomain=Discrete-time  SampleTime=dt  IntegratorMethod=Forward Euler  FilterMethod=Forward Euler  ControllerParametersSource=internal  P=TASRateErr2VRate  I=TASRateErrInt2VRate  D=0  UseFilter=on  N=100  TunerSelectOption=Transfer Function Based (PID Tuner App)  InitialConditionSource=internal  InitialConditionForIntegrator=0  InitialConditionForFilter=0  DifferentiatorICPrevScaledInput=0  ExternalReset=level  TrackingMode=off  Kt=1  LimitOutput=off  UpperSaturationLimit=10  LowerSaturationLimit=-10  LinearizeAsGain=on  AntiWindupMode=none  Kb=1  POutMin=[]  POutMax=[]  IOutMin=[]  IOutMax=[]  DOutMin=[]  DOutMax=[]  NOutMin=[]  NOutMax=[]  SumOutMin=[]  SumOutMax=[]  SaturationOutMin=[]  SaturationOutMax=[]  PParamMin=[]  PParamMax=[]  IParamMin=[]  IParamMax=[]  DParamMin=[]  DParamMax=[]  NParamMin=[]  NParamMax=[]  KbParamMin=[]  KbParamMax=[]  KtParamMin=[]  KtParamMax=[]  KbOutMin=[]  KbOutMax=[]  KtOutMin=[]  KtOutMax=[]  IntegratorOutMin=[]  IntegratorOutMax=[]  FilterOutMin=[]  FilterOutMax=[]  SumI1OutMin=[]  SumI1OutMax=[]  SumI2OutMin=[]  SumI2OutMax=[]  SumI3OutMin=[]  SumI3OutMax=[]  SumI4OutMin=[]  SumI4OutMax=[]  SumDOutMin=[]  SumDOutMax=[]  DifferentiatorOutMin=[]  DifferentiatorOutMax=[]  FilterDiffOutCoefMin=[]  FilterDiffOutCoefMax=[]  ReciprocalOutMin=[]  ReciprocalOutMax=[]  SumDenOutMin=[]  SumDenOutMax=[]  SumNumOutMin=[]  SumNumOutMax=[]  DivideOutMin=[]  DivideOutMax=[]  IntegratorContinuousStateAttributes=''  IntegratorStateMustResolveToSignalObject=off  IntegratorRTWStateStorageClass=Auto  FilterContinuousStateAttributes=''  FilterStateMustResolveToSignalObject=off  FilterRTWStateStorageClass=Auto  ParallelPVariant=InternalParameters  IdealPVariant=Disabled  IVariant=InternalParameters  DVariant=InternalParameters  IntegratorVariant=Discrete  SatVariant=Disabled  AWVariant=Passthrough  PCopyVariant=Disabled  TRVariant=Disabled  FdbkBlocksVariant=Forward  IdealPFdbkVariant=Disabled  SatFdbkVariant=Disabled  DerivativeFilterVariant=ForwardEulerFilter  NVariant=InternalParameters  NCopyVariant=Disabled  FilterICVariant=InternalICsFilter  IntegratorICVariant=InternalICs  ExternalResetVariant=ExternalReset  TRSumVariant=Passthrough  SumFdbkVariant=Disabled  SumVariant=Sum_PID
  Saturation Dynamic : simulink/Discontinuities/Saturation Dynamic  OutMin=[]  OutMax=[]  OutDataTypeStr=Inherit: Same as second input  OutDataType=fixdt(1, 16)  OutScaling=2^-10  DoSatur=off
  Subsystem : Subsystem
  Sum : Sum  Inputs=|-+
  hdotCmd : Outport
  wires:
  VdotCmd/1 -> Sum/1
  Feedback Bus/1 -> Bus Selector/1
  Bus Selector/1 -> Sum/2  "<Vdot_mps2>"
  Sum/1 -> PID Controller/1
  PID Controller/1 -> Saturation Dynamic/2
  Saturation Dynamic/1 -> hdotCmd/1  "Sim.VRateCmd(airspeed)"
  Bus Selector/2 -> Subsystem/1(V)  "<V_mps>"
  Subsystem/1(hdotMax) -> Saturation Dynamic/1
  Subsystem/2("hdotMin ") -> Saturation Dynamic/3
  Vcmd/1 -> Subsystem/2(Vcmd)
  OR/1 -> PID Controller/2
  Bus Selector/3 -> Compare To Constant/1  "<apMode>"
  [ApGlobal] -> NOT/1
  Compare To Constant/1 -> OR/1
  NOT/1 -> OR/2
  [Flag_TAS_Priority] -> NOT1/1
  NOT1/1 -> OR/3

== system Lib_Piccolo/Altitude Rate to Pitch Command/Integrator ==
  In : Inport
  Reset : Inport  Port=2
  Init : Inport  Port=3
  Enable : EnablePort
  Discrete-Time Integrator : DiscreteIntegrator  IntegratorMethod=Integration: Backward Euler  ExternalReset=level  InitialConditionSource=external  SampleTime=-1  LimitOutput=on  UpperSaturationLimit=PitchMax  LowerSaturationLimit=-PitchMax  ICPrevOutput=DiscIntNeverNeededParam  ICPrevScaledInput=DiscIntNeverNeededParam
  Out : Outport
  wires:
  In/1 -> Discrete-Time Integrator/1
  Discrete-Time Integrator/1 -> Out/1
  Reset/1 -> Discrete-Time Integrator/2
  Init/1 -> Discrete-Time Integrator/3
